simulink model "codeur_hamming"  (R2023b)
settings: Solver=FixedStepDiscrete  StartTime=0.0  StopTime=111  FixedStep=1  RelTol=1e-3
settings Model: Creator=e2507477  LastModifiedBy=e2507477

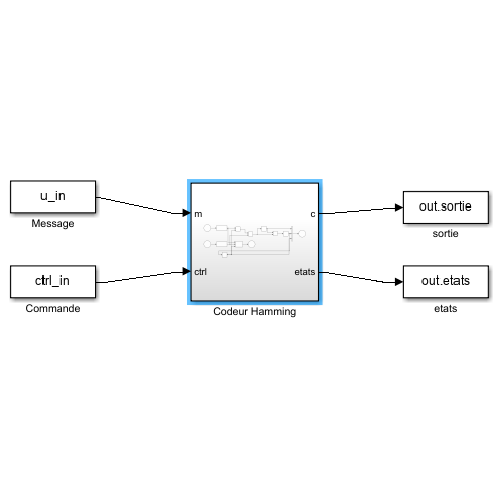
[thumbnail: Simulink's stored preview of the top-level diagram]
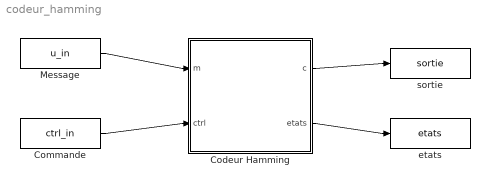
== system codeur_hamming ==
  Codeur Hamming : Subsystem
  Commande : FromWorkspace  VariableName=ctrl_in  SampleTime=1  Interpolate=off  OutputAfterFinalValue=Holding final value
  Message : FromWorkspace  VariableName=u_in  SampleTime=1  Interpolate=off  OutputAfterFinalValue=Holding final value
  etats : ToWorkspace  VariableName=etats  SampleTime=-1
  sortie : ToWorkspace  VariableName=sortie  SampleTime=-1
  wires:
  Message/1 -> Codeur Hamming/1(m)
  Commande/1 -> Codeur Hamming/2(ctrl)
  Codeur Hamming/1(c) -> sortie/1
  Codeur Hamming/2(etats) -> etats/1

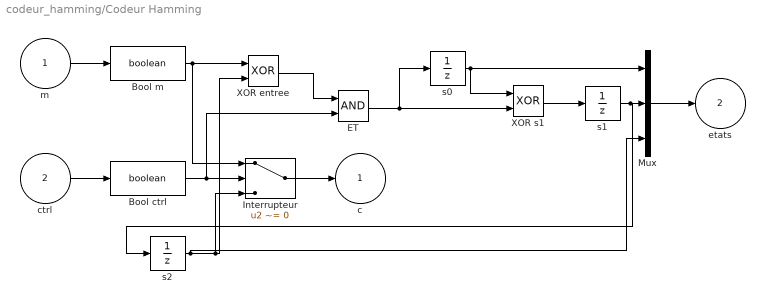
== system codeur_hamming/Codeur Hamming ==
  m : Inport
  ctrl : Inport  Port=2
  Bool ctrl : DataTypeConversion  OutDataTypeStr=boolean  SaturateOnIntegerOverflow=off  RndMeth=Floor
  Bool m : DataTypeConversion  OutDataTypeStr=boolean  SaturateOnIntegerOverflow=off  RndMeth=Floor
  ET : Logic  AllPortsSameDT=off  OutDataTypeStr=boolean
  Interrupteur : Switch  Criteria=u2 ~= 0  SaturateOnIntegerOverflow=off  InputSameDT=off
  Mux : Mux  Inputs=3
  XOR entree : Logic  Operator=XOR  AllPortsSameDT=off  OutDataTypeStr=boolean
  XOR s1 : Logic  Operator=XOR  AllPortsSameDT=off  OutDataTypeStr=boolean
  s0 : UnitDelay  HasFrameUpgradeWarning=on
  s1 : UnitDelay  HasFrameUpgradeWarning=on
  s2 : UnitDelay  HasFrameUpgradeWarning=on
  c : Outport
  etats : Outport  Port=2
  wires:
  m/1 -> Bool m/1
  ctrl/1 -> Bool ctrl/1
  Bool m/1 -> XOR entree/1, Interrupteur/1
  Bool ctrl/1 -> ET/2, Interrupteur/2
  Interrupteur/1 -> c/1
  s2/1 -> XOR entree/2, Interrupteur/3, Mux/3
  XOR entree/1 -> ET/1
  ET/1 -> XOR s1/2, s0/1
  s0/1 -> Mux/1, XOR s1/1
  s1/1 -> s2/1, Mux/2
  XOR s1/1 -> s1/1
  Mux/1 -> etats/1
